simulink model "youBot_Arm_before_acceleration_test"  (R2024a)
settings: Solver=ode15s  StartTime=0.0  StopTime=3.3  MaxStep=1e-2  RelTol=1e-3  AbsTol=1e-4
model workspace: external: MATLAB File youBot_DataFile.m (data not in the file)
undefined symbols (not defined in the file): Extr_Data_LinkHoles, Qt, sigbuilder_block, smiData, X, Y, YBT_Par, Z
libraries: sm_lib x193, nesl_utility x130, fl_lib x53, simulink x13, Parts_Lib x10, MyMath_lib x8, Motor_Lib x5, Contact_Forces_Lib x4, ee_lib x2, sdl_lib x2
(part 2 of 8)

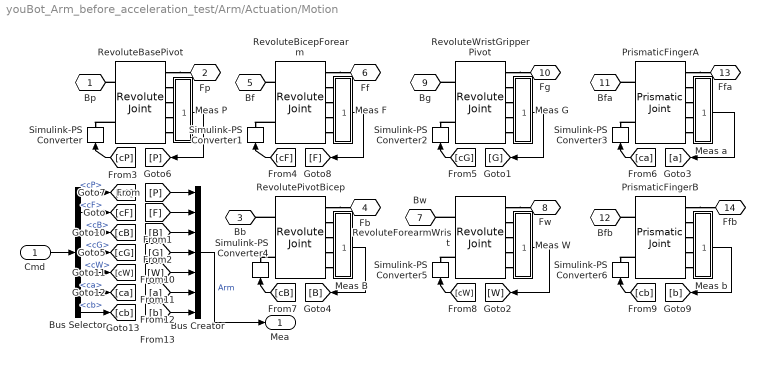
== system youBot_Arm_before_acceleration_test/Arm/Actuation/Motion ==
  Cmd : Inport
  Bus Creator : BusCreator  Inputs=7
  Bus Selector : BusSelector  OutputSignals=cP,cF,cB,cG,cW,ca,cb
  Meas B : Subsystem
      mask Display: disp('m')
  Meas F : Subsystem
      mask Display: disp('m')
  Meas G : Subsystem
      mask Display: disp('m')
  Meas P : Subsystem  Tag=CustomStyle
      mask Display: disp('m')
  Meas W : Subsystem
      mask Display: disp('m')
  Meas a : Subsystem
      mask Display: disp('m')
  Meas b : Subsystem
      mask Display: disp('m')
  PrismaticFingerA : sm_lib/Joints/Prismatic Joint  JointMode=Normal  CompositeWrenchDir=FollowerOnBase  CompositeWrenchFrame=BaseFrame  SenseConstraintForce=on  SenseConstraintTorque=off  SenseTotalForce=off  SenseTotalTorque=off  PositionTargetSpecify=on  PositionTargetPriority=Low  PositionTargetValue=smiData.PrismaticJoint(2).Pz.Pos  PositionTargetValueUnits=m  VelocityTargetSpecify=off  VelocityTargetPriority=High  VelocityTargetValue=0  VelocityTargetValueUnits=m/s  EquilibriumPosition=0  EquilibriumPositionUnits=m  SpringStiffness=0  SpringStiffnessUnits=N/m  DampingCoefficient=0  DampingCoefficientUnits=N/(m/s)  LowerLimitSpecify=off  LowerLimitBound=-1  LowerLimitBoundUnits=m  LowerLimitStiffness=1e6  LowerLimitStiffnessUnits=N/m  LowerLimitDamping=1e3  LowerLimitDampingUnits=N/(m/s)  LowerLimitTransitionRegionWidth=1e-4  LowerLimitTransitionRegionWidthUnits=m  UpperLimitSpecify=off  UpperLimitBound=1  UpperLimitBoundUnits=m  UpperLimitStiffness=1e6  UpperLimitStiffnessUnits=N/m  UpperLimitDamping=1e3  UpperLimitDampingUnits=N/(m/s)  UpperLimitTransitionRegionWidth=1e-4  UpperLimitTransitionRegionWidthUnits=m  TorqueActuationMode=ComputedTorque  MotionActuationMode=InputMotion  SensePosition=on  SenseVelocity=on  SenseAcceleration=off  SenseTorqueForce=on  SenseLowerLimitTorqueForce=off  SenseUpperLimitTorqueForce=off
  PrismaticFingerB : sm_lib/Joints/Prismatic Joint  JointMode=Normal  CompositeWrenchDir=FollowerOnBase  CompositeWrenchFrame=BaseFrame  SenseConstraintForce=on  SenseConstraintTorque=off  SenseTotalForce=off  SenseTotalTorque=off  PositionTargetSpecify=on  PositionTargetPriority=Low  PositionTargetValue=smiData.PrismaticJoint(1).Pz.Pos  PositionTargetValueUnits=m  VelocityTargetSpecify=off  VelocityTargetPriority=High  VelocityTargetValue=0  VelocityTargetValueUnits=m/s  EquilibriumPosition=0  EquilibriumPositionUnits=m  SpringStiffness=0  SpringStiffnessUnits=N/m  DampingCoefficient=0  DampingCoefficientUnits=N/(m/s)  LowerLimitSpecify=off  LowerLimitBound=-1  LowerLimitBoundUnits=m  LowerLimitStiffness=1e6  LowerLimitStiffnessUnits=N/m  LowerLimitDamping=1e3  LowerLimitDampingUnits=N/(m/s)  LowerLimitTransitionRegionWidth=1e-4  LowerLimitTransitionRegionWidthUnits=m  UpperLimitSpecify=off  UpperLimitBound=1  UpperLimitBoundUnits=m  UpperLimitStiffness=1e6  UpperLimitStiffnessUnits=N/m  UpperLimitDamping=1e3  UpperLimitDampingUnits=N/(m/s)  UpperLimitTransitionRegionWidth=1e-4  UpperLimitTransitionRegionWidthUnits=m  TorqueActuationMode=ComputedTorque  MotionActuationMode=InputMotion  SensePosition=on  SenseVelocity=on  SenseAcceleration=off  SenseTorqueForce=on  SenseLowerLimitTorqueForce=off  SenseUpperLimitTorqueForce=off
  RevoluteBasePivot : sm_lib/Joints/Revolute Joint  JointMode=Normal  CompositeWrenchDir=FollowerOnBase  CompositeWrenchFrame=BaseFrame  SenseConstraintForce=on  SenseConstraintTorque=off  SenseTotalForce=off  SenseTotalTorque=off  PositionTargetSpecify=on  PositionTargetPriority=Low  PositionTargetValue=smiData.RevoluteJoint(3).Rz.Pos  PositionTargetValueUnits=deg  VelocityTargetSpecify=off  VelocityTargetPriority=High  VelocityTargetValue=0  VelocityTargetValueUnits=deg/s  EquilibriumPosition=0  EquilibriumPositionUnits=rad  SpringStiffness=0  SpringStiffnessUnits=N*m/rad  DampingCoefficient=YBT_Par.Pivot.Motor.friction  DampingCoefficientUnits=N*m/(rad/s)  LowerLimitSpecify=off  LowerLimitBound=-90  LowerLimitBoundUnits=deg  LowerLimitStiffness=1e4  LowerLimitStiffnessUnits=N*m/deg  LowerLimitDamping=10  LowerLimitDampingUnits=N*m/(deg/s)  LowerLimitTransitionRegionWidth=0.1  LowerLimitTransitionRegionWidthUnits=deg  UpperLimitSpecify=off  UpperLimitBound=90  UpperLimitBoundUnits=deg  UpperLimitStiffness=1e4  UpperLimitStiffnessUnits=N*m/deg  UpperLimitDamping=10  UpperLimitDampingUnits=N*m/(deg/s)  UpperLimitTransitionRegionWidth=0.1  UpperLimitTransitionRegionWidthUnits=deg  TorqueActuationMode=ComputedTorque  MotionActuationMode=InputMotion  SensePosition=on  SenseVelocity=on  SenseAcceleration=off  SenseTorqueForce=on  SenseLowerLimitTorqueForce=off  SenseUpperLimitTorqueForce=off
  RevoluteBicepForearm : sm_lib/Joints/Revolute Joint  JointMode=Normal  CompositeWrenchDir=FollowerOnBase  CompositeWrenchFrame=BaseFrame  SenseConstraintForce=on  SenseConstraintTorque=off  SenseTotalForce=off  SenseTotalTorque=off  PositionTargetSpecify=on  PositionTargetPriority=Low  PositionTargetValue=smiData.RevoluteJoint(2).Rz.Pos  PositionTargetValueUnits=deg  VelocityTargetSpecify=off  VelocityTargetPriority=High  VelocityTargetValue=0  VelocityTargetValueUnits=deg/s  EquilibriumPosition=0  EquilibriumPositionUnits=rad  SpringStiffness=0  SpringStiffnessUnits=N*m/rad  DampingCoefficient=YBT_Par.Forearm.Motor.friction  DampingCoefficientUnits=N*m/(rad/s)  LowerLimitSpecify=off  LowerLimitBound=-90  LowerLimitBoundUnits=deg  LowerLimitStiffness=1e4  LowerLimitStiffnessUnits=N*m/deg  LowerLimitDamping=10  LowerLimitDampingUnits=N*m/(deg/s)  LowerLimitTransitionRegionWidth=0.1  LowerLimitTransitionRegionWidthUnits=deg  UpperLimitSpecify=off  UpperLimitBound=90  UpperLimitBoundUnits=deg  UpperLimitStiffness=1e4  UpperLimitStiffnessUnits=N*m/deg  UpperLimitDamping=10  UpperLimitDampingUnits=N*m/(deg/s)  UpperLimitTransitionRegionWidth=0.1  UpperLimitTransitionRegionWidthUnits=deg  TorqueActuationMode=ComputedTorque  MotionActuationMode=InputMotion  SensePosition=on  SenseVelocity=on  SenseAcceleration=off  SenseTorqueForce=on  SenseLowerLimitTorqueForce=off  SenseUpperLimitTorqueForce=off
  RevoluteForearmWrist : sm_lib/Joints/Revolute Joint  JointMode=Normal  CompositeWrenchDir=FollowerOnBase  CompositeWrenchFrame=BaseFrame  SenseConstraintForce=on  SenseConstraintTorque=off  SenseTotalForce=off  SenseTotalTorque=off  PositionTargetSpecify=on  PositionTargetPriority=Low  PositionTargetValue=smiData.RevoluteJoint(5).Rz.Pos  PositionTargetValueUnits=deg  VelocityTargetSpecify=off  VelocityTargetPriority=High  VelocityTargetValue=0  VelocityTargetValueUnits=deg/s  EquilibriumPosition=0  EquilibriumPositionUnits=rad  SpringStiffness=0  SpringStiffnessUnits=N*m/rad  DampingCoefficient=YBT_Par.Wrist.Motor.friction  DampingCoefficientUnits=N*m/(rad/s)  LowerLimitSpecify=off  LowerLimitBound=-90  LowerLimitBoundUnits=deg  LowerLimitStiffness=1e4  LowerLimitStiffnessUnits=N*m/deg  LowerLimitDamping=10  LowerLimitDampingUnits=N*m/(deg/s)  LowerLimitTransitionRegionWidth=0.1  LowerLimitTransitionRegionWidthUnits=deg  UpperLimitSpecify=off  UpperLimitBound=90  UpperLimitBoundUnits=deg  UpperLimitStiffness=1e4  UpperLimitStiffnessUnits=N*m/deg  UpperLimitDamping=10  UpperLimitDampingUnits=N*m/(deg/s)  UpperLimitTransitionRegionWidth=0.1  UpperLimitTransitionRegionWidthUnits=deg  TorqueActuationMode=ComputedTorque  MotionActuationMode=InputMotion  SensePosition=on  SenseVelocity=on  SenseAcceleration=off  SenseTorqueForce=on  SenseLowerLimitTorqueForce=off  SenseUpperLimitTorqueForce=off
  RevolutePivotBicep : sm_lib/Joints/Revolute Joint  JointMode=Normal  CompositeWrenchDir=FollowerOnBase  CompositeWrenchFrame=BaseFrame  SenseConstraintForce=on  SenseConstraintTorque=off  SenseTotalForce=off  SenseTotalTorque=off  PositionTargetSpecify=on  PositionTargetPriority=Low  PositionTargetValue=smiData.RevoluteJoint(1).Rz.Pos  PositionTargetValueUnits=deg  VelocityTargetSpecify=off  VelocityTargetPriority=High  VelocityTargetValue=0  VelocityTargetValueUnits=deg/s  EquilibriumPosition=0  EquilibriumPositionUnits=rad  SpringStiffness=0  SpringStiffnessUnits=N*m/rad  DampingCoefficient=YBT_Par.Bicep.Motor.friction  DampingCoefficientUnits=N*m/(rad/s)  LowerLimitSpecify=off  LowerLimitBound=-90  LowerLimitBoundUnits=deg  LowerLimitStiffness=1e4  LowerLimitStiffnessUnits=N*m/deg  LowerLimitDamping=10  LowerLimitDampingUnits=N*m/(deg/s)  LowerLimitTransitionRegionWidth=0.1  LowerLimitTransitionRegionWidthUnits=deg  UpperLimitSpecify=off  UpperLimitBound=90  UpperLimitBoundUnits=deg  UpperLimitStiffness=1e4  UpperLimitStiffnessUnits=N*m/deg  UpperLimitDamping=10  UpperLimitDampingUnits=N*m/(deg/s)  UpperLimitTransitionRegionWidth=0.1  UpperLimitTransitionRegionWidthUnits=deg  TorqueActuationMode=ComputedTorque  MotionActuationMode=InputMotion  SensePosition=on  SenseVelocity=on  SenseAcceleration=off  SenseTorqueForce=on  SenseLowerLimitTorqueForce=off  SenseUpperLimitTorqueForce=off
  RevoluteWristGripperPivot : sm_lib/Joints/Revolute Joint  JointMode=Normal  CompositeWrenchDir=FollowerOnBase  CompositeWrenchFrame=BaseFrame  SenseConstraintForce=on  SenseConstraintTorque=off  SenseTotalForce=off  SenseTotalTorque=off  PositionTargetSpecify=on  PositionTargetPriority=Low  PositionTargetValue=smiData.RevoluteJoint(4).Rz.Pos  PositionTargetValueUnits=deg  VelocityTargetSpecify=off  VelocityTargetPriority=High  VelocityTargetValue=0  VelocityTargetValueUnits=deg/s  EquilibriumPosition=0  EquilibriumPositionUnits=rad  SpringStiffness=0  SpringStiffnessUnits=N*m/rad  DampingCoefficient=YBT_Par.Gripper.Motor.friction  DampingCoefficientUnits=N*m/(rad/s)  LowerLimitSpecify=off  LowerLimitBound=-90  LowerLimitBoundUnits=deg  LowerLimitStiffness=1e4  LowerLimitStiffnessUnits=N*m/deg  LowerLimitDamping=10  LowerLimitDampingUnits=N*m/(deg/s)  LowerLimitTransitionRegionWidth=0.1  LowerLimitTransitionRegionWidthUnits=deg  UpperLimitSpecify=off  UpperLimitBound=90  UpperLimitBoundUnits=deg  UpperLimitStiffness=1e4  UpperLimitStiffnessUnits=N*m/deg  UpperLimitDamping=10  UpperLimitDampingUnits=N*m/(deg/s)  UpperLimitTransitionRegionWidth=0.1  UpperLimitTransitionRegionWidthUnits=deg  TorqueActuationMode=ComputedTorque  MotionActuationMode=InputMotion  SensePosition=on  SenseVelocity=on  SenseAcceleration=off  SenseTorqueForce=on  SenseLowerLimitTorqueForce=off  SenseUpperLimitTorqueForce=off
  Simulink-PS Converter{,1..2,4..5} (5 alike) : nesl_utility/Simulink-PS Converter  Tag=CustomStyle  PhysicalDomain=network_engine_domain  SubClassName=ps_input  LeftPortType=input  RightPortType=output  PseudoPeriodic=off  Frequencies=[]  NoiseDistribution=none  NoiseParameters=[]  Unit=deg  AffineConversion=off  FilteringAndDerivatives=filter  SimscapeFilterOrder=2  InputFilterTimeConstant=0.005  UdotUserProvided=1
  Simulink-PS Converter3 : nesl_utility/Simulink-PS Converter  Tag=CustomStyle  PhysicalDomain=network_engine_domain  SubClassName=ps_input  LeftPortType=input  RightPortType=output  PseudoPeriodic=off  Frequencies=[]  NoiseDistribution=none  NoiseParameters=[]  Unit=mm  AffineConversion=off  FilteringAndDerivatives=filter  SimscapeFilterOrder=2  InputFilterTimeConstant=0.005  UdotUserProvided=1
  Simulink-PS Converter6 : nesl_utility/Simulink-PS Converter  Tag=CustomStyle  PhysicalDomain=network_engine_domain  SubClassName=ps_input  LeftPortType=input  RightPortType=output  PseudoPeriodic=off  Frequencies=[]  NoiseDistribution=none  NoiseParameters=[]  Unit=mm  AffineConversion=off  FilteringAndDerivatives=filter  SimscapeFilterOrder=2  InputFilterTimeConstant=0.005  UdotUserProvided=1
  Bp : PMIOPort  Side=Right
  Fp : PMIOPort  Port=2  Side=Right
  Bb : PMIOPort  Port=3  Side=Right
  Fb : PMIOPort  Port=4  Side=Right
  Bf : PMIOPort  Port=5  Side=Right
  Ff : PMIOPort  Port=6  Side=Right
  Bw : PMIOPort  Port=7  Side=Right
  Fw : PMIOPort  Port=8  Side=Right
  Bg : PMIOPort  Port=9  Side=Right
  Fg : PMIOPort  Port=10  Side=Right
  Bfa : PMIOPort  Port=11  Side=Right
  Bfb : PMIOPort  Port=12  Side=Right
  Ffa : PMIOPort  Port=13  Side=Right
  Ffb : PMIOPort  Port=14  Side=Right
  Mea : Outport  VectorParamsAs1DForOutWhenUnconnected=off
  wires:
  Bus Creator/1 -> Mea/1  "Arm"
  Cmd/1 -> Bus Selector/1
  [cP] -> Simulink-PS Converter/1
  Bus Selector/1 -> [cP]  "<cP>"
  Meas F/1(F) -> [F]
  [cF] -> Simulink-PS Converter1/1
  [cG] -> Simulink-PS Converter2/1
  [ca] -> Simulink-PS Converter3/1
  Meas B/1(B) -> [B]
  [cB] -> Simulink-PS Converter4/1
  Meas W/1(W) -> [W]
  [cW] -> Simulink-PS Converter5/1
  Meas b/1(b) -> [b]
  [cb] -> Simulink-PS Converter6/1
  Bus Selector/2 -> [cF]  "<cF>"
  Bus Selector/3 -> [cB]  "<cB>"
  Bus Selector/4 -> [cG]  "<cG>"
  Bus Selector/5 -> [cW]  "<cW>"
  Bus Selector/6 -> [ca]  "<ca>"
  Bus Selector/7 -> [cb]  "<cb>"
  [P] -> Bus Creator/1
  [F] -> Bus Creator/2
  [B] -> Bus Creator/3
  [G] -> Bus Creator/4
  [W] -> Bus Creator/5
  [a] -> Bus Creator/6
  [b] -> Bus Creator/7
  Meas P/1(P) -> [P]
  Meas G/1(G) -> [G]
  Meas a/1(a) -> [a]
  connections:
  RevoluteForearmWrist/RConn1 -- Fw/RConn1
  RevolutePivotBicep/LConn1 -- Bb/RConn1
  RevoluteForearmWrist/LConn1 -- Bw/RConn1
  RevoluteBicepForearm/RConn1 -- Ff/RConn1
  RevolutePivotBicep/RConn1 -- Fb/RConn1
  RevoluteBicepForearm/LConn1 -- Bf/RConn1
  RevoluteWristGripperPivot/LConn1 -- Bg/RConn1
  RevoluteWristGripperPivot/RConn1 -- Fg/RConn1
  PrismaticFingerA/RConn1 -- Ffa/RConn1
  PrismaticFingerA/LConn1 -- Bfa/RConn1
  PrismaticFingerB/LConn1 -- Bfb/RConn1
  PrismaticFingerB/RConn1 -- Ffb/RConn1
  RevoluteBasePivot/LConn1 -- Bp/RConn1
  RevoluteBasePivot/RConn1 -- Fp/RConn1
  RevoluteBasePivot/LConn2 -- Simulink-PS Converter/RConn1
  RevoluteBicepForearm/LConn2 -- Simulink-PS Converter1/RConn1
  RevoluteWristGripperPivot/LConn2 -- Simulink-PS Converter2/RConn1
  PrismaticFingerA/LConn2 -- Simulink-PS Converter3/RConn1
  RevolutePivotBicep/LConn2 -- Simulink-PS Converter4/RConn1
  RevoluteForearmWrist/LConn2 -- Simulink-PS Converter5/RConn1
  PrismaticFingerB/LConn2 -- Simulink-PS Converter6/RConn1
  RevoluteBasePivot/RConn2 -- Meas P/LConn1
  RevoluteBasePivot/RConn3 -- Meas P/LConn2
  RevoluteBasePivot/RConn4 -- Meas P/LConn3
  RevoluteBicepForearm/RConn2 -- Meas F/LConn1
  RevoluteBicepForearm/RConn3 -- Meas F/LConn2
  RevoluteBicepForearm/RConn4 -- Meas F/LConn3
  RevolutePivotBicep/RConn2 -- Meas B/LConn1
  RevolutePivotBicep/RConn3 -- Meas B/LConn2
  RevolutePivotBicep/RConn4 -- Meas B/LConn3
  RevoluteWristGripperPivot/RConn2 -- Meas G/LConn1
  RevoluteWristGripperPivot/RConn3 -- Meas G/LConn2
  RevoluteWristGripperPivot/RConn4 -- Meas G/LConn3
  RevoluteForearmWrist/RConn2 -- Meas W/LConn1
  RevoluteForearmWrist/RConn3 -- Meas W/LConn2
  RevoluteForearmWrist/RConn4 -- Meas W/LConn3
  PrismaticFingerB/RConn2 -- Meas b/LConn1
  PrismaticFingerB/RConn3 -- Meas b/LConn2
  PrismaticFingerB/RConn4 -- Meas b/LConn3
  PrismaticFingerA/RConn2 -- Meas a/LConn1
  PrismaticFingerA/RConn3 -- Meas a/LConn2
  PrismaticFingerA/RConn4 -- Meas a/LConn3
  RevoluteBicepForearm/RConn5 -- Meas F/LConn4
  RevoluteWristGripperPivot/RConn5 -- Meas G/LConn4
  RevoluteForearmWrist/RConn5 -- Meas W/LConn4
  PrismaticFingerB/RConn5 -- Meas b/LConn4
  PrismaticFingerA/RConn5 -- Meas a/LConn4
  RevoluteBasePivot/RConn5 -- Meas P/LConn4
  RevolutePivotBicep/RConn5 -- Meas B/LConn4

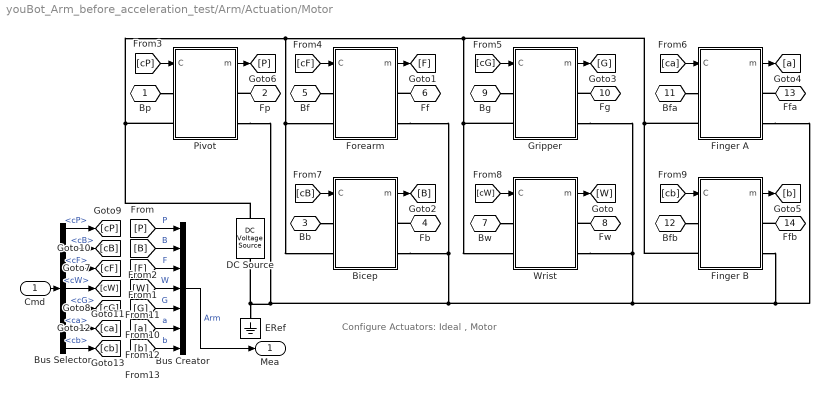
== system youBot_Arm_before_acceleration_test/Arm/Actuation/Motor ==
  note: Configure Actuators: Ideal , Motor
  Cmd : Inport
  Bicep : Subsystem  Variant=on  VariantControlMode=label  LabelModeActiveChoice=Ideal
      settings: AttributesFormatString=%<ActiveVariant>
      mask Display:
      | blk = youBot_Arm_activeVariantBlock(gcb);
      | eval(get_param(blk, 'MaskDisplay'));
  Bus Creator : BusCreator  Inputs=7
  Bus Selector : BusSelector  OutputSignals=cP,cB,cF,cW,cG,ca,cb
  DC Source : fl_lib/Electrical/Electrical Sources/DC Voltage Source  v0=24 V
  ERef : fl_lib/Electrical/Electrical Elements/Electrical Reference
  Finger A : Subsystem
      mask Display: image('youBot_Arm_Actuation_MotorPris_Ideal_IMAGE.jpg');
  Finger B : Subsystem
      mask Display: image('youBot_Arm_Actuation_MotorPris_Ideal_IMAGE.jpg');
  Forearm : Subsystem  Variant=on  VariantControlMode=label  LabelModeActiveChoice=Ideal
      settings: AttributesFormatString=%<ActiveVariant>
      mask Display:
      | blk = youBot_Arm_activeVariantBlock(gcb);
      | eval(get_param(blk, 'MaskDisplay'));
  Gripper : Subsystem  Variant=on  VariantControlMode=label  LabelModeActiveChoice=Ideal
      settings: AttributesFormatString=%<ActiveVariant>
      mask Display:
      | blk = youBot_Arm_activeVariantBlock(gcb);
      | eval(get_param(blk, 'MaskDisplay'));
  Pivot : Subsystem  Variant=on  VariantControlMode=label  LabelModeActiveChoice=Ideal
      settings: AttributesFormatString=%<ActiveVariant>
      mask Display:
      | blk = youBot_Arm_activeVariantBlock(gcb);
      | eval(get_param(blk, 'MaskDisplay'));
  Wrist : Subsystem  Variant=on  VariantControlMode=label  LabelModeActiveChoice=Ideal
      settings: AttributesFormatString=%<ActiveVariant>
      mask Display:
      | blk = youBot_Arm_activeVariantBlock(gcb);
      | eval(get_param(blk, 'MaskDisplay'));
  Bp : PMIOPort  Side=Right
  Fp : PMIOPort  Port=2  Side=Right
  Bb : PMIOPort  Port=3  Side=Right
  Fb : PMIOPort  Port=4  Side=Right
  Bf : PMIOPort  Port=5  Side=Right
  Ff : PMIOPort  Port=6  Side=Right
  Bw : PMIOPort  Port=7  Side=Right
  Fw : PMIOPort  Port=8  Side=Right
  Bg : PMIOPort  Port=9  Side=Right
  Fg : PMIOPort  Port=10  Side=Right
  Bfa : PMIOPort  Port=11  Side=Right
  Bfb : PMIOPort  Port=12  Side=Right
  Ffa : PMIOPort  Port=13  Side=Right
  Ffb : PMIOPort  Port=14  Side=Right
  Mea : Outport  VectorParamsAs1DForOutWhenUnconnected=off
  wires:
  Pivot/1(m) -> [P]
  Finger B/1(m) -> [b]
  Finger A/1(m) -> [a]
  Gripper/1(m) -> [G]
  Wrist/1(m) -> [W]
  Bicep/1(m) -> [B]
  Forearm/1(m) -> [F]
  Bus Creator/1 -> Mea/1  "Arm"
  Cmd/1 -> Bus Selector/1
  Bus Selector/1 -> [cP]  "<cP>"
  Bus Selector/3 -> [cF]  "<cF>"
  Bus Selector/2 -> [cB]  "<cB>"
  Bus Selector/5 -> [cG]  "<cG>"
  Bus Selector/4 -> [cW]  "<cW>"
  Bus Selector/6 -> [ca]  "<ca>"
  Bus Selector/7 -> [cb]  "<cb>"
  [P] -> Bus Creator/1  "P"
  [B] -> Bus Creator/2  "B"
  [F] -> Bus Creator/3  "F"
  [G] -> Bus Creator/5  "G"
  [W] -> Bus Creator/4  "W"
  [a] -> Bus Creator/6  "a"
  [b] -> Bus Creator/7  "b"
  [cF] -> Forearm/1(C)
  [ca] -> Finger A/1(C)
  [cG] -> Gripper/1(C)
  [cP] -> Pivot/1(C)
  [cB] -> Bicep/1(C)
  [cW] -> Wrist/1(C)
  [cb] -> Finger B/1(C)
  connections:
  Fp/RConn1 -- Pivot/RConn1
  Bp/RConn1 -- Pivot/LConn1
  Ffb/RConn1 -- Finger B/RConn1
  Bfb/RConn1 -- Finger B/LConn1
  Bfa/RConn1 -- Finger A/LConn1
  Ffa/RConn1 -- Finger A/RConn1
  Fg/RConn1 -- Gripper/RConn1
  Bg/RConn1 -- Gripper/LConn1
  Gripper/LConn2 -- Finger B/LConn2 -- Finger A/LConn2 -- Bicep/LConn2 -- Forearm/LConn2 -- DC Source/LConn1 -- Pivot/LConn2 -- Wrist/LConn2
  Bf/RConn1 -- Forearm/LConn1
  Fb/RConn1 -- Bicep/RConn1
  Ff/RConn1 -- Forearm/RConn1
  Bw/RConn1 -- Wrist/LConn1
  Forearm/RConn2 -- Bicep/RConn2 -- Gripper/RConn2 -- Wrist/RConn2 -- Finger B/RConn2 -- Finger A/RConn2 -- Pivot/RConn2 -- DC Source/RConn1 -- ERef/LConn1
  Bb/RConn1 -- Bicep/LConn1
  Fw/RConn1 -- Wrist/RConn1

== system youBot_Arm_before_acceleration_test/Arm/Base/Base_1_RIGID ==
  ReferenceFrame : sm_lib/Frames and Transforms/Reference Frame
  Solid : sm_lib/Body Elements/File Solid  ExtGeomFileName=Base.step  UnitType=FromFile  ExtGeomFileUnits=m  StepReaderType=HEX  ExportConvexHullGeometry=off  InertiaType=Custom  BasedOnType=Density  Density=1000  DensityUnits=kg/m^3  Mass=smiData.Solid(11).mass  MassUnits=kg  CenterOfMass=smiData.Solid(11).CoM  CenterOfMassUnits=m  MomentsOfInertia=smiData.Solid(11).MoI  MomentsOfInertiaUnits=kg*m^2  ProductsOfInertia=smiData.Solid(11).PoI  ProductsOfInertiaUnits=kg*m^2  GraphicType=FromGeometry  MarkerShape=Sphere  MarkerSize=10  GraphicVisPropType=SimpleVisualProperties  GraphicDiffuseColor=smiData.Solid(11).color  GraphicOpacity=smiData.Solid(11).opacity  GraphicSpecularColor=[0.5 0.5 0.5 1.0]  GraphicAmbientColor=[0.15 0.15 0.15 1.0]  GraphicEmissiveColor=[0.0 0.0 0.0 1.0]  GraphicShininess=75  DoExposeReferenceFrame=on  SerializedFrames=<Frames/>
  Transform : sm_lib/Frames and Transforms/Rigid Transform  RotationMethod=ArbitraryAxis  FollAlignAxisA=+X  BaseAlignAxisA=+Y  FollAlignAxisB=+Y  BaseAlignAxisB=+Z  RotationStandardAxis=+Z  RotationAngle=smiData.RigidTransform(21).angle  RotationAngleUnits=rad  RotationArbitraryAxis=smiData.RigidTransform(21).axis  RotationSequenceAxes=FollowerAxes  RotationSequence=XYX  RotationSequenceAngles=[0 0 0]  RotationSequenceAnglesUnits=deg  RotationMatrix=[1 0 0; 0 1 0; 0 0 1]  Quaternion=[1 0 0 0]  TranslationMethod=Cartesian  TranslationCartesianOffset=smiData.RigidTransform(21).translation  TranslationCartesianOffsetUnits=m  TranslationStandardAxis=+Z  TranslationStandardOffset=0  TranslationStandardOffsetUnits=m  TranslationROffset=0  TranslationROffsetUnits=m  TranslationThetaOffset=0  TranslationThetaOffsetUnits=deg  TranslationZOffset=0  TranslationZOffsetUnits=m
  F1 : PMIOPort  Side=Left
  F : PMIOPort  Port=2  Side=Right
  connections:
  Solid/RConn1 -- ReferenceFrame/RConn1 -- Transform/LConn1 -- F1/RConn1
  Transform/RConn1 -- F/RConn1

== system youBot_Arm_before_acceleration_test/Arm/Bicep/Bicep_1_RIGID ==
  ReferenceFrame : sm_lib/Frames and Transforms/Reference Frame
  Solid : sm_lib/Body Elements/File Solid  ExtGeomFileName=Bicep.step  UnitType=FromFile  ExtGeomFileUnits=m  StepReaderType=HEX  ExportConvexHullGeometry=off  InertiaType=Custom  BasedOnType=Density  Density=1000  DensityUnits=kg/m^3  Mass=smiData.Solid(3).mass  MassUnits=kg  CenterOfMass=smiData.Solid(3).CoM  CenterOfMassUnits=m  MomentsOfInertia=smiData.Solid(3).MoI  MomentsOfInertiaUnits=kg*m^2  ProductsOfInertia=smiData.Solid(3).PoI  ProductsOfInertiaUnits=kg*m^2  GraphicType=FromGeometry  MarkerShape=Sphere  MarkerSize=10  GraphicVisPropType=SimpleVisualProperties  GraphicDiffuseColor=smiData.Solid(3).color  GraphicOpacity=smiData.Solid(3).opacity  GraphicSpecularColor=[0.5 0.5 0.5 1.0]  GraphicAmbientColor=[0.15 0.15 0.15 1.0]  GraphicEmissiveColor=[0.0 0.0 0.0 1.0]  GraphicShininess=75  DoExposeReferenceFrame=on  SerializedFrames=<Frames/>
  Transform : sm_lib/Frames and Transforms/Rigid Transform  RotationMethod=ArbitraryAxis  FollAlignAxisA=+X  BaseAlignAxisA=+Y  FollAlignAxisB=+Y  BaseAlignAxisB=+Z  RotationStandardAxis=+Z  RotationAngle=smiData.RigidTransform(18).angle  RotationAngleUnits=rad  RotationArbitraryAxis=smiData.RigidTransform(18).axis  RotationSequenceAxes=FollowerAxes  RotationSequence=XYX  RotationSequenceAngles=[0 0 0]  RotationSequenceAnglesUnits=deg  RotationMatrix=[1 0 0; 0 1 0; 0 0 1]  Quaternion=[1 0 0 0]  TranslationMethod=Cartesian  TranslationCartesianOffset=smiData.RigidTransform(18).translation  TranslationCartesianOffsetUnits=m  TranslationStandardAxis=+Z  TranslationStandardOffset=0  TranslationStandardOffsetUnits=m  TranslationROffset=0  TranslationROffsetUnits=m  TranslationThetaOffset=0  TranslationThetaOffsetUnits=deg  TranslationZOffset=0  TranslationZOffsetUnits=m
  Transform1 : sm_lib/Frames and Transforms/Rigid Transform  RotationMethod=ArbitraryAxis  FollAlignAxisA=+X  BaseAlignAxisA=+Y  FollAlignAxisB=+Y  BaseAlignAxisB=+Z  RotationStandardAxis=+Z  RotationAngle=smiData.RigidTransform(19).angle  RotationAngleUnits=rad  RotationArbitraryAxis=smiData.RigidTransform(19).axis  RotationSequenceAxes=FollowerAxes  RotationSequence=XYX  RotationSequenceAngles=[0 0 0]  RotationSequenceAnglesUnits=deg  RotationMatrix=[1 0 0; 0 1 0; 0 0 1]  Quaternion=[1 0 0 0]  TranslationMethod=Cartesian  TranslationCartesianOffset=smiData.RigidTransform(19).translation  TranslationCartesianOffsetUnits=m  TranslationStandardAxis=+Z  TranslationStandardOffset=0  TranslationStandardOffsetUnits=m  TranslationROffset=0  TranslationROffsetUnits=m  TranslationThetaOffset=0  TranslationThetaOffsetUnits=deg  TranslationZOffset=0  TranslationZOffsetUnits=m
  F : PMIOPort  Side=Left
  F1 : PMIOPort  Port=2  Side=Right
  connections:
  Solid/RConn1 -- ReferenceFrame/RConn1 -- Transform/LConn1 -- Transform1/LConn1
  Transform/RConn1 -- F/RConn1
  Transform1/RConn1 -- F1/RConn1

== system youBot_Arm_before_acceleration_test/Arm/Environment/Conveyors ==
  Belt : Inport
  Belt In : Subsystem  Tag=PublishSubsystem
      mask Display: image('youBot_Arm_Conveyors_IMAGE.jpg');
  Belt Out : Subsystem
      mask Display: image('youBot_Arm_Conveyors_IMAGE.jpg');
  Bus Creator : BusCreator  Inputs=2
  Bus Selector : BusSelector  OutputSignals=Belt In On,Belt Out On
  Transform Belt In : sm_lib/Frames and Transforms/Rigid Transform  RotationMethod=StandardAxis  FollAlignAxisA=+X  BaseAlignAxisA=+Y  FollAlignAxisB=+Y  BaseAlignAxisB=+Z  RotationStandardAxis=+Z  RotationAngle=-90  RotationAngleUnits=deg  RotationArbitraryAxis=[0 0 1]  RotationSequenceAxes=FollowerAxes  RotationSequence=XYX  RotationSequenceAngles=[0 0 0]  RotationSequenceAnglesUnits=deg  RotationMatrix=[1 0 0; 0 1 0; 0 0 1]  Quaternion=[1 0 0 0]  TranslationMethod=Cartesian  TranslationCartesianOffset=YBT_Par.BeltIn.offset  TranslationCartesianOffsetUnits=m  TranslationStandardAxis=+Y  TranslationStandardOffset=0  TranslationStandardOffsetUnits=m  TranslationROffset=0  TranslationROffsetUnits=m  TranslationThetaOffset=0  TranslationThetaOffsetUnits=deg  TranslationZOffset=0  TranslationZOffsetUnits=m
  Transform Belt Out : sm_lib/Frames and Transforms/Rigid Transform  RotationMethod=StandardAxis  FollAlignAxisA=+X  BaseAlignAxisA=+Y  FollAlignAxisB=+Y  BaseAlignAxisB=+Z  RotationStandardAxis=+Z  RotationAngle=180  RotationAngleUnits=deg  RotationArbitraryAxis=[0 0 1]  RotationSequenceAxes=FollowerAxes  RotationSequence=XYX  RotationSequenceAngles=[0 0 0]  RotationSequenceAnglesUnits=deg  RotationMatrix=[1 0 0; 0 1 0; 0 0 1]  Quaternion=[1 0 0 0]  TranslationMethod=Cartesian  TranslationCartesianOffset=YBT_Par.BeltOut.offset  TranslationCartesianOffsetUnits=m  TranslationStandardAxis=+Y  TranslationStandardOffset=0  TranslationStandardOffsetUnits=m  TranslationROffset=0  TranslationROffsetUnits=m  TranslationThetaOffset=0  TranslationThetaOffsetUnits=deg  TranslationZOffset=0  TranslationZOffsetUnits=m
  Floor : PMIOPort  Side=Left
  Box : PMIOPort  Port=2  Side=Right
  Sensors : Outport  VectorParamsAs1DForOutWhenUnconnected=off
  wires:
  Bus Selector/1 -> Belt In/1(On)  "<Belt In On>"
  Belt/1 -> Bus Selector/1
  Bus Selector/2 -> Belt Out/1(On)  "<Belt Out On>"
  Belt In/1(Sensors) -> Bus Creator/1
  Belt Out/1(Sensors) -> Bus Creator/2
  Bus Creator/1 -> Sensors/1  "Belts"
  connections:
  Floor/RConn1 -- Transform Belt Out/LConn1 -- Transform Belt In/LConn1
  Box/RConn1 -- Belt Out/RConn1 -- Belt In/RConn1
  Transform Belt In/RConn1 -- Belt In/LConn1
  Belt Out/LConn1 -- Transform Belt Out/RConn1

== system youBot_Arm_before_acceleration_test/Arm/Environment/EE Signals ==
  Mux : Mux  Inputs=3
  PS-Simulink Converter : nesl_utility/PS-Simulink Converter  PhysicalDomain=network_engine_domain  SubClassName=ps_output  LeftPortType=input  RightPortType=output  PseudoPeriodic=off  Frequencies=[]  VectorFormat=1-D array  Unit=1  AffineConversion=off
  PS-Simulink Converter1 : nesl_utility/PS-Simulink Converter  PhysicalDomain=network_engine_domain  SubClassName=ps_output  LeftPortType=input  RightPortType=output  PseudoPeriodic=off  Frequencies=[]  VectorFormat=1-D array  Unit=1  AffineConversion=off
  PS-Simulink Converter2 : nesl_utility/PS-Simulink Converter  PhysicalDomain=network_engine_domain  SubClassName=ps_output  LeftPortType=input  RightPortType=output  PseudoPeriodic=off  Frequencies=[]  VectorFormat=1-D array  Unit=1  AffineConversion=off
  x : PMIOPort  Side=Left
  y : PMIOPort  Port=2  Side=Left
  z : PMIOPort  Port=3  Side=Left
  xyz : Outport  VectorParamsAs1DForOutWhenUnconnected=off
  wires:
  PS-Simulink Converter1/1 -> Mux/2
  PS-Simulink Converter2/1 -> Mux/3
  PS-Simulink Converter/1 -> Mux/1
  Mux/1 -> xyz/1
  connections:
  PS-Simulink Converter2/LConn1 -- z/RConn1
  PS-Simulink Converter/LConn1 -- x/RConn1
  PS-Simulink Converter1/LConn1 -- y/RConn1

== system youBot_Arm_before_acceleration_test/Arm/Environment/Floor ==
  Floor : sm_lib/Body Elements/Brick Solid  Commented=on  BrickDimensions=[YBT_Par.Floor.r*2 YBT_Par.Floor.r*2 YBT_Par.Floor.d]  BrickDimensionsUnits=m  ExportEntireGeometry=off  InertiaType=CalculateFromGeometry  BasedOnType=Density  Density=1000  DensityUnits=kg/m^3  Mass=1  MassUnits=kg  CenterOfMass=[0 0 0]  CenterOfMassUnits=m  MomentsOfInertia=[1 1 1]  MomentsOfInertiaUnits=kg*m^2  ProductsOfInertia=[1 1 1]  ProductsOfInertiaUnits=kg*m^2  GraphicType=FromGeometry  MarkerShape=Sphere  MarkerSize=10  GraphicVisPropType=SimpleVisualProperties  GraphicDiffuseColor=[0.8 0.8 0.8]  GraphicOpacity=1  GraphicSpecularColor=[0.5 0.5 0.5 1.0]  GraphicAmbientColor=[0.15 0.15 0.15 1.0]  GraphicEmissiveColor=[0.0 0.0 0.0 1.0]  GraphicShininess=75  DoExposeReferenceFrame=on  SerializedFrames=<Frames><Frame><Id>Frame1</Id><Value><Name>T</Name><Origin><Source>GeometricFeature</Source><FeatureName>+z surface</FeatureName></Origin><PrimaryAxis><DefinedDirection>+Z</DefinedDirection><Source>ReferenceFrame</Source><SourceDirection>+Z</SourceDirection><FeatureName></FeatureName></PrimaryAxis><SecondaryAxis><DefinedDirection>+X</DefinedDirection><Source>ReferenceFrame</Source><SourceDirection>+X</SourceDirection><FeatureName></FeatureName></SecondaryAxis></Value></Frame></Frames>
  T : PMIOPort  Side=Left
  connections:
  Floor/LConn1 -- T/RConn1

== system youBot_Arm_before_acceleration_test/Arm/Environment/Gripper Force ==
  Damper : Subsystem  VariantControl=Damper
      mask Display: image('youBot_Arm_Gripper_Force_Damper_IMAGE.jpg');
  Payload : Subsystem  VariantControl=Payload
      mask Display: image('youBot_Arm_Gripper_Force_Payload_IMAGE.jpg');
  Penalty : Subsystem  Tag=PublishSubsystem  VariantControl=Penalty
      mask Display: image('youBot_Arm_Gripper_Force_Penalty_IMAGE.jpg');
  Fa : PMIOPort  Side=Right
  Bfa : PMIOPort  Port=2  Side=Left
  E : PMIOPort  Port=3  Side=Right
  Fb : PMIOPort  Port=4  Side=Right
  Bfb : PMIOPort  Port=5  Side=Left

== system youBot_Arm_before_acceleration_test/Arm/Environment/Load ==
  Box : Subsystem  VariantControl=Box
      mask Display: image('youBot_Arm_Box_IMAGE.jpg');
  None : Subsystem  VariantControl=None
      mask Display: disp(' ')
  Fa : PMIOPort  Side=Right
  Ctr : PMIOPort  Port=2  Side=Left
  Fb : PMIOPort  Port=3  Side=Right
  W : PMIOPort  Port=4  Side=Left

== system youBot_Arm_before_acceleration_test/Arm/Finger A/Finger_A_1_RIGID ==
  ReferenceFrame : sm_lib/Frames and Transforms/Reference Frame
  Solid : sm_lib/Body Elements/File Solid  ExtGeomFileName=Finger A.step  UnitType=FromFile  ExtGeomFileUnits=m  StepReaderType=HEX  ExportConvexHullGeometry=off  InertiaType=Custom  BasedOnType=Density  Density=1000  DensityUnits=kg/m^3  Mass=smiData.Solid(2).mass  MassUnits=kg  CenterOfMass=smiData.Solid(2).CoM  CenterOfMassUnits=m  MomentsOfInertia=smiData.Solid(2).MoI  MomentsOfInertiaUnits=kg*m^2  ProductsOfInertia=smiData.Solid(2).PoI  ProductsOfInertiaUnits=kg*m^2  GraphicType=FromGeometry  MarkerShape=Sphere  MarkerSize=10  GraphicVisPropType=SimpleVisualProperties  GraphicDiffuseColor=smiData.Solid(2).color  GraphicOpacity=smiData.Solid(2).opacity  GraphicSpecularColor=[0.5 0.5 0.5 1.0]  GraphicAmbientColor=[0.15 0.15 0.15 1.0]  GraphicEmissiveColor=[0.0 0.0 0.0 1.0]  GraphicShininess=75  DoExposeReferenceFrame=on  SerializedFrames=<Frames><Frame><Id>Frame1</Id><Value><Name>Face</Name><Origin><Source>GeometricFeature</Source><FeatureName>planar surface 32</FeatureName></Origin><PrimaryAxis><DefinedDirection>+Z</DefinedDirection><Source>ReferenceFrame</Source><SourceDirection>+X</SourceDirection><FeatureName></FeatureName></PrimaryAxis><SecondaryAxis><DefinedDirection>+X</DefinedDirection><Source>ReferenceFrame</Source><SourceDirection>+Y</SourceDirection><FeatureName></FeatureName></SecondaryAxis></Value></Frame></Frames>
  Transform : sm_lib/Frames and Transforms/Rigid Transform  RotationMethod=ArbitraryAxis  FollAlignAxisA=+X  BaseAlignAxisA=+Y  FollAlignAxisB=+Y  BaseAlignAxisB=+Z  RotationStandardAxis=+Z  RotationAngle=smiData.RigidTransform(42).angle  RotationAngleUnits=rad  RotationArbitraryAxis=smiData.RigidTransform(42).axis  RotationSequenceAxes=FollowerAxes  RotationSequence=XYX  RotationSequenceAngles=[0 0 0]  RotationSequenceAnglesUnits=deg  RotationMatrix=[1 0 0; 0 1 0; 0 0 1]  Quaternion=[1 0 0 0]  TranslationMethod=Cartesian  TranslationCartesianOffset=smiData.RigidTransform(42).translation  TranslationCartesianOffsetUnits=m  TranslationStandardAxis=+Z  TranslationStandardOffset=0  TranslationStandardOffsetUnits=m  TranslationROffset=0  TranslationROffsetUnits=m  TranslationThetaOffset=0  TranslationThetaOffsetUnits=deg  TranslationZOffset=0  TranslationZOffsetUnits=m
  Transform Contact Ctr : sm_lib/Frames and Transforms/Rigid Transform  RotationMethod=None  FollAlignAxisA=+X  BaseAlignAxisA=+Y  FollAlignAxisB=+Y  BaseAlignAxisB=+Z  RotationStandardAxis=+Z  RotationAngle=0.0  RotationAngleUnits=deg  RotationArbitraryAxis=[0 0 1]  RotationSequenceAxes=FollowerAxes  RotationSequence=XYX  RotationSequenceAngles=[0 0 0]  RotationSequenceAnglesUnits=deg  RotationMatrix=[1 0 0; 0 1 0; 0 0 1]  Quaternion=[1 0 0 0]  TranslationMethod=StandardAxis  TranslationCartesianOffset=[0 0 0]  TranslationCartesianOffsetUnits=m  TranslationStandardAxis=+Y  TranslationStandardOffset=YBT_Par.Finger.Con.yoffset  TranslationStandardOffsetUnits=m  TranslationROffset=0  TranslationROffsetUnits=m  TranslationThetaOffset=0  TranslationThetaOffsetUnits=deg  TranslationZOffset=0  TranslationZOffsetUnits=m
  F : PMIOPort  Side=Left
  Face : PMIOPort  Port=2  Side=Right
  connections:
  ReferenceFrame/RConn1 -- Solid/RConn1 -- Transform/LConn1
  Transform/RConn1 -- F/RConn1
  Transform Contact Ctr/LConn1 -- Solid/LConn1
  Face/RConn1 -- Transform Contact Ctr/RConn1

== system youBot_Arm_before_acceleration_test/Arm/Finger B/Finger_B_1_RIGID ==
  ReferenceFrame : sm_lib/Frames and Transforms/Reference Frame
  Solid : sm_lib/Body Elements/File Solid  ExtGeomFileName=Finger B.step  UnitType=FromFile  ExtGeomFileUnits=m  StepReaderType=HEX  ExportConvexHullGeometry=off  InertiaType=Custom  BasedOnType=Density  Density=1000  DensityUnits=kg/m^3  Mass=smiData.Solid(7).mass  MassUnits=kg  CenterOfMass=smiData.Solid(7).CoM  CenterOfMassUnits=m  MomentsOfInertia=smiData.Solid(7).MoI  MomentsOfInertiaUnits=kg*m^2  ProductsOfInertia=smiData.Solid(7).PoI  ProductsOfInertiaUnits=kg*m^2  GraphicType=FromGeometry  MarkerShape=Sphere  MarkerSize=10  GraphicVisPropType=SimpleVisualProperties  GraphicDiffuseColor=smiData.Solid(7).color  GraphicOpacity=smiData.Solid(7).opacity  GraphicSpecularColor=[0.5 0.5 0.5 1.0]  GraphicAmbientColor=[0.15 0.15 0.15 1.0]  GraphicEmissiveColor=[0.0 0.0 0.0 1.0]  GraphicShininess=75  DoExposeReferenceFrame=on  SerializedFrames=<Frames><Frame><Id>Frame1</Id><Value><Name>Face</Name><Origin><Source>GeometricFeature</Source><FeatureName>planar surface 34</FeatureName></Origin><PrimaryAxis><DefinedDirection>+Z</DefinedDirection><Source>ReferenceFrame</Source><SourceDirection>-X</SourceDirection><FeatureName></FeatureName></PrimaryAxis><SecondaryAxis><DefinedDirection>+X</DefinedDirection><Source>ReferenceFrame</Source><SourceDirection>-Y</SourceDirection><FeatureName></FeatureName></SecondaryAxis></Value></Frame></Frames>
  Transform : sm_lib/Frames and Transforms/Rigid Transform  RotationMethod=ArbitraryAxis  FollAlignAxisA=+X  BaseAlignAxisA=+Y  FollAlignAxisB=+Y  BaseAlignAxisB=+Z  RotationStandardAxis=+Z  RotationAngle=smiData.RigidTransform(2).angle  RotationAngleUnits=rad  RotationArbitraryAxis=smiData.RigidTransform(2).axis  RotationSequenceAxes=FollowerAxes  RotationSequence=XYX  RotationSequenceAngles=[0 0 0]  RotationSequenceAnglesUnits=deg  RotationMatrix=[1 0 0; 0 1 0; 0 0 1]  Quaternion=[1 0 0 0]  TranslationMethod=Cartesian  TranslationCartesianOffset=smiData.RigidTransform(2).translation  TranslationCartesianOffsetUnits=m  TranslationStandardAxis=+Z  TranslationStandardOffset=0  TranslationStandardOffsetUnits=m  TranslationROffset=0  TranslationROffsetUnits=m  TranslationThetaOffset=0  TranslationThetaOffsetUnits=deg  TranslationZOffset=0  TranslationZOffsetUnits=m
  Transform Contact Ctr : sm_lib/Frames and Transforms/Rigid Transform  RotationMethod=None  FollAlignAxisA=+X  BaseAlignAxisA=+Y  FollAlignAxisB=+Y  BaseAlignAxisB=+Z  RotationStandardAxis=+Z  RotationAngle=0.0  RotationAngleUnits=deg  RotationArbitraryAxis=[0 0 1]  RotationSequenceAxes=FollowerAxes  RotationSequence=XYX  RotationSequenceAngles=[0 0 0]  RotationSequenceAnglesUnits=deg  RotationMatrix=[1 0 0; 0 1 0; 0 0 1]  Quaternion=[1 0 0 0]  TranslationMethod=StandardAxis  TranslationCartesianOffset=[0 0 0]  TranslationCartesianOffsetUnits=m  TranslationStandardAxis=+Y  TranslationStandardOffset=YBT_Par.Finger.Con.yoffset  TranslationStandardOffsetUnits=m  TranslationROffset=0  TranslationROffsetUnits=m  TranslationThetaOffset=0  TranslationThetaOffsetUnits=deg  TranslationZOffset=0  TranslationZOffsetUnits=m
  F : PMIOPort  Side=Left
  Face : PMIOPort  Port=2  Side=Right
  connections:
  ReferenceFrame/RConn1 -- Transform/LConn1 -- Solid/RConn1
  Transform/RConn1 -- F/RConn1
  Transform Contact Ctr/LConn1 -- Solid/LConn1
  Face/RConn1 -- Transform Contact Ctr/RConn1

== system youBot_Arm_before_acceleration_test/Arm/Forearm/Forearm_1_RIGID ==
  ReferenceFrame : sm_lib/Frames and Transforms/Reference Frame
  Solid : sm_lib/Body Elements/File Solid  ExtGeomFileName=Forearm.step  UnitType=FromFile  ExtGeomFileUnits=m  StepReaderType=HEX  ExportConvexHullGeometry=off  InertiaType=Custom  BasedOnType=Density  Density=1000  DensityUnits=kg/m^3  Mass=smiData.Solid(21).mass  MassUnits=kg  CenterOfMass=smiData.Solid(21).CoM  CenterOfMassUnits=m  MomentsOfInertia=smiData.Solid(21).MoI  MomentsOfInertiaUnits=kg*m^2  ProductsOfInertia=smiData.Solid(21).PoI  ProductsOfInertiaUnits=kg*m^2  GraphicType=FromGeometry  MarkerShape=Sphere  MarkerSize=10  GraphicVisPropType=SimpleVisualProperties  GraphicDiffuseColor=smiData.Solid(21).color  GraphicOpacity=smiData.Solid(21).opacity  GraphicSpecularColor=[0.5 0.5 0.5 1.0]  GraphicAmbientColor=[0.15 0.15 0.15 1.0]  GraphicEmissiveColor=[0.0 0.0 0.0 1.0]  GraphicShininess=75  DoExposeReferenceFrame=on  SerializedFrames=<Frames/>
  Transform : sm_lib/Frames and Transforms/Rigid Transform  RotationMethod=ArbitraryAxis  FollAlignAxisA=+X  BaseAlignAxisA=+Y  FollAlignAxisB=+Y  BaseAlignAxisB=+Z  RotationStandardAxis=+Z  RotationAngle=smiData.RigidTransform(20).angle  RotationAngleUnits=rad  RotationArbitraryAxis=smiData.RigidTransform(20).axis  RotationSequenceAxes=FollowerAxes  RotationSequence=XYX  RotationSequenceAngles=[0 0 0]  RotationSequenceAnglesUnits=deg  RotationMatrix=[1 0 0; 0 1 0; 0 0 1]  Quaternion=[1 0 0 0]  TranslationMethod=Cartesian  TranslationCartesianOffset=smiData.RigidTransform(20).translation  TranslationCartesianOffsetUnits=m  TranslationStandardAxis=+Z  TranslationStandardOffset=0  TranslationStandardOffsetUnits=m  TranslationROffset=0  TranslationROffsetUnits=m  TranslationThetaOffset=0  TranslationThetaOffsetUnits=deg  TranslationZOffset=0  TranslationZOffsetUnits=m
  Transform1 : sm_lib/Frames and Transforms/Rigid Transform  RotationMethod=ArbitraryAxis  FollAlignAxisA=+X  BaseAlignAxisA=+Y  FollAlignAxisB=+Y  BaseAlignAxisB=+Z  RotationStandardAxis=+Z  RotationAngle=smiData.RigidTransform(29).angle  RotationAngleUnits=rad  RotationArbitraryAxis=smiData.RigidTransform(29).axis  RotationSequenceAxes=FollowerAxes  RotationSequence=XYX  RotationSequenceAngles=[0 0 0]  RotationSequenceAnglesUnits=deg  RotationMatrix=[1 0 0; 0 1 0; 0 0 1]  Quaternion=[1 0 0 0]  TranslationMethod=Cartesian  TranslationCartesianOffset=smiData.RigidTransform(29).translation  TranslationCartesianOffsetUnits=m  TranslationStandardAxis=+Z  TranslationStandardOffset=0  TranslationStandardOffsetUnits=m  TranslationROffset=0  TranslationROffsetUnits=m  TranslationThetaOffset=0  TranslationThetaOffsetUnits=deg  TranslationZOffset=0  TranslationZOffsetUnits=m
  Transform2 : sm_lib/Frames and Transforms/Rigid Transform  RotationMethod=ArbitraryAxis  FollAlignAxisA=+X  BaseAlignAxisA=+Y  FollAlignAxisB=+Y  BaseAlignAxisB=+Z  RotationStandardAxis=+Z  RotationAngle=smiData.RigidTransform(47).angle  RotationAngleUnits=rad  RotationArbitraryAxis=smiData.RigidTransform(47).axis  RotationSequenceAxes=FollowerAxes  RotationSequence=XYX  RotationSequenceAngles=[0 0 0]  RotationSequenceAnglesUnits=deg  RotationMatrix=[1 0 0; 0 1 0; 0 0 1]  Quaternion=[1 0 0 0]  TranslationMethod=Cartesian  TranslationCartesianOffset=smiData.RigidTransform(47).translation  TranslationCartesianOffsetUnits=m  TranslationStandardAxis=+Z  TranslationStandardOffset=0  TranslationStandardOffsetUnits=m  TranslationROffset=0  TranslationROffsetUnits=m  TranslationThetaOffset=0  TranslationThetaOffsetUnits=deg  TranslationZOffset=0  TranslationZOffsetUnits=m
  F2 : PMIOPort  Side=Left
  F : PMIOPort  Port=2  Side=Left
  F1 : PMIOPort  Port=3  Side=Right
  connections:
  Solid/RConn1 -- ReferenceFrame/RConn1 -- Transform/LConn1 -- Transform1/LConn1 -- Transform2/LConn1
  Transform/RConn1 -- F/RConn1
  Transform1/RConn1 -- F1/RConn1
  Transform2/RConn1 -- F2/RConn1

== system youBot_Arm_before_acceleration_test/Arm/Forearm/Forearm_Black_Inlay_1_RIGID ==
  ReferenceFrame : sm_lib/Frames and Transforms/Reference Frame
  Solid : sm_lib/Body Elements/File Solid  ExtGeomFileName=Forearm Black Inlay.step  UnitType=FromFile  ExtGeomFileUnits=m  StepReaderType=HEX  ExportConvexHullGeometry=off  InertiaType=Custom  BasedOnType=Density  Density=1000  DensityUnits=kg/m^3  Mass=smiData.Solid(6).mass  MassUnits=kg  CenterOfMass=smiData.Solid(6).CoM  CenterOfMassUnits=m  MomentsOfInertia=smiData.Solid(6).MoI  MomentsOfInertiaUnits=kg*m^2  ProductsOfInertia=smiData.Solid(6).PoI  ProductsOfInertiaUnits=kg*m^2  GraphicType=FromGeometry  MarkerShape=Sphere  MarkerSize=10  GraphicVisPropType=SimpleVisualProperties  GraphicDiffuseColor=smiData.Solid(6).color  GraphicOpacity=smiData.Solid(6).opacity  GraphicSpecularColor=[0.5 0.5 0.5 1.0]  GraphicAmbientColor=[0.15 0.15 0.15 1.0]  GraphicEmissiveColor=[0.0 0.0 0.0 1.0]  GraphicShininess=75  DoExposeReferenceFrame=on  SerializedFrames=<Frames/>
  Transform : sm_lib/Frames and Transforms/Rigid Transform  RotationMethod=ArbitraryAxis  FollAlignAxisA=+X  BaseAlignAxisA=+Y  FollAlignAxisB=+Y  BaseAlignAxisB=+Z  RotationStandardAxis=+Z  RotationAngle=smiData.RigidTransform(48).angle  RotationAngleUnits=rad  RotationArbitraryAxis=smiData.RigidTransform(48).axis  RotationSequenceAxes=FollowerAxes  RotationSequence=XYX  RotationSequenceAngles=[0 0 0]  RotationSequenceAnglesUnits=deg  RotationMatrix=[1 0 0; 0 1 0; 0 0 1]  Quaternion=[1 0 0 0]  TranslationMethod=Cartesian  TranslationCartesianOffset=smiData.RigidTransform(48).translation  TranslationCartesianOffsetUnits=m  TranslationStandardAxis=+Z  TranslationStandardOffset=0  TranslationStandardOffsetUnits=m  TranslationROffset=0  TranslationROffsetUnits=m  TranslationThetaOffset=0  TranslationThetaOffsetUnits=deg  TranslationZOffset=0  TranslationZOffsetUnits=m
  F : PMIOPort  Side=Left
  connections:
  Solid/RConn1 -- ReferenceFrame/RConn1 -- Transform/LConn1
  Transform/RConn1 -- F/RConn1

== system youBot_Arm_before_acceleration_test/Arm/Gripper/Electronics_Board_1_RIGID ==
  ReferenceFrame : sm_lib/Frames and Transforms/Reference Frame
  Solid : sm_lib/Body Elements/File Solid  ExtGeomFileName=Electronics Board.step  UnitType=FromFile  ExtGeomFileUnits=m  StepReaderType=HEX  ExportConvexHullGeometry=off  InertiaType=Custom  BasedOnType=Density  Density=1000  DensityUnits=kg/m^3  Mass=smiData.Solid(17).mass  MassUnits=kg  CenterOfMass=smiData.Solid(17).CoM  CenterOfMassUnits=m  MomentsOfInertia=smiData.Solid(17).MoI  MomentsOfInertiaUnits=kg*m^2  ProductsOfInertia=smiData.Solid(17).PoI  ProductsOfInertiaUnits=kg*m^2  GraphicType=FromGeometry  MarkerShape=Sphere  MarkerSize=10  GraphicVisPropType=SimpleVisualProperties  GraphicDiffuseColor=smiData.Solid(17).color  GraphicOpacity=smiData.Solid(17).opacity  GraphicSpecularColor=[0.5 0.5 0.5 1.0]  GraphicAmbientColor=[0.15 0.15 0.15 1.0]  GraphicEmissiveColor=[0.0 0.0 0.0 1.0]  GraphicShininess=75  DoExposeReferenceFrame=on  SerializedFrames=<Frames/>
  Transform : sm_lib/Frames and Transforms/Rigid Transform  RotationMethod=ArbitraryAxis  FollAlignAxisA=+X  BaseAlignAxisA=+Y  FollAlignAxisB=+Y  BaseAlignAxisB=+Z  RotationStandardAxis=+Z  RotationAngle=smiData.RigidTransform(14).angle  RotationAngleUnits=rad  RotationArbitraryAxis=smiData.RigidTransform(14).axis  RotationSequenceAxes=FollowerAxes  RotationSequence=XYX  RotationSequenceAngles=[0 0 0]  RotationSequenceAnglesUnits=deg  RotationMatrix=[1 0 0; 0 1 0; 0 0 1]  Quaternion=[1 0 0 0]  TranslationMethod=Cartesian  TranslationCartesianOffset=smiData.RigidTransform(14).translation  TranslationCartesianOffsetUnits=m  TranslationStandardAxis=+Z  TranslationStandardOffset=0  TranslationStandardOffsetUnits=m  TranslationROffset=0  TranslationROffsetUnits=m  TranslationThetaOffset=0  TranslationThetaOffsetUnits=deg  TranslationZOffset=0  TranslationZOffsetUnits=m
  Transform1 : sm_lib/Frames and Transforms/Rigid Transform  RotationMethod=ArbitraryAxis  FollAlignAxisA=+X  BaseAlignAxisA=+Y  FollAlignAxisB=+Y  BaseAlignAxisB=+Z  RotationStandardAxis=+Z  RotationAngle=smiData.RigidTransform(31).angle  RotationAngleUnits=rad  RotationArbitraryAxis=smiData.RigidTransform(31).axis  RotationSequenceAxes=FollowerAxes  RotationSequence=XYX  RotationSequenceAngles=[0 0 0]  RotationSequenceAnglesUnits=deg  RotationMatrix=[1 0 0; 0 1 0; 0 0 1]  Quaternion=[1 0 0 0]  TranslationMethod=Cartesian  TranslationCartesianOffset=smiData.RigidTransform(31).translation  TranslationCartesianOffsetUnits=m  TranslationStandardAxis=+Z  TranslationStandardOffset=0  TranslationStandardOffsetUnits=m  TranslationROffset=0  TranslationROffsetUnits=m  TranslationThetaOffset=0  TranslationThetaOffsetUnits=deg  TranslationZOffset=0  TranslationZOffsetUnits=m
  F : PMIOPort  Side=Left
  F1 : PMIOPort  Port=2  Side=Left
  connections:
  Solid/RConn1 -- ReferenceFrame/RConn1 -- Transform/LConn1 -- Transform1/LConn1
  Transform/RConn1 -- F/RConn1
  Transform1/RConn1 -- F1/RConn1
